simulink model "Balancing_Robot_Rob_Tracking"  (R2024b)
settings: Solver=VariableStepAuto  StartTime=0.0  StopTime=30  RelTol=1e-3
undefined symbols (not defined in the file): body, C12, C_filter, DiscIntNeverNeededParam, drv, dspblkCoreblockFVToolHelper, Fv_pr, g, g22, gbox, gcbh, K_Rob_LQR, Ki_calc, M11, M12_const, M22, mot, ms22g, Nu, Nx, sens, T, ua2tau, wheel
settings Model: Creator=liliy  LastModifiedBy=liliy

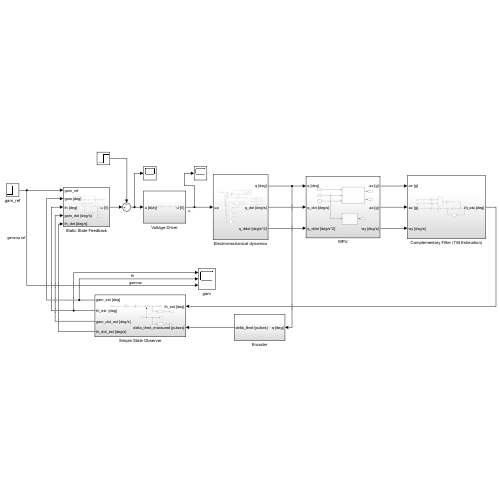
[thumbnail: Simulink's stored preview of the top-level diagram]
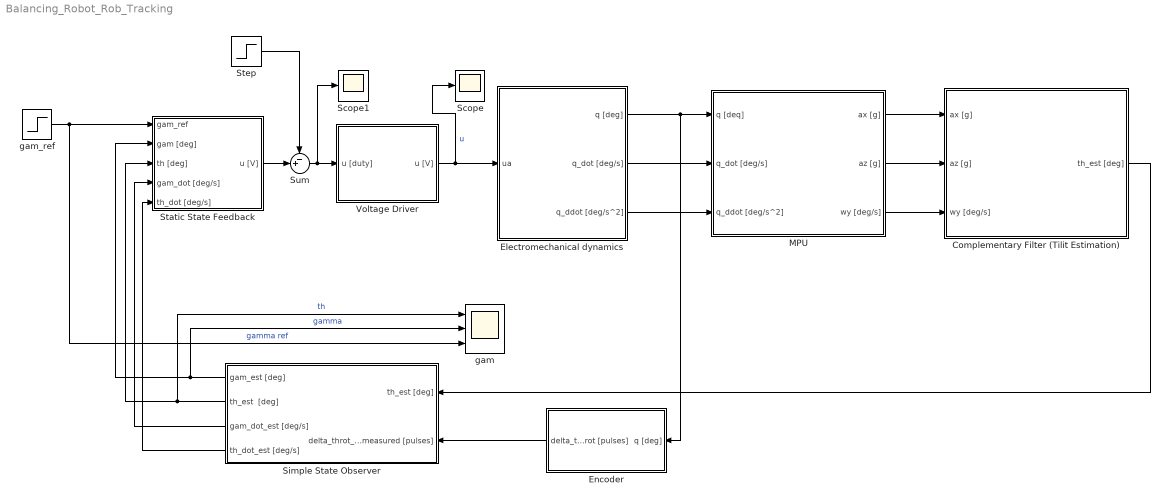
== system Balancing_Robot_Rob_Tracking ==
  Complementary Filter (Tilit Estimation) : Subsystem
  Electromechanical dynamics : Subsystem
  Encoder : Subsystem
  MPU : Subsystem
  Scope : Scope
  Scope1 : Scope
  Simple State Observer : Subsystem
  Static State Feedback : Subsystem
  Step : Step  Time=10  After=5/drv.duty2V  SampleTime=0
  Sum : Sum  Inputs=-+|
  Voltage Driver : Subsystem
  gam : Scope  NumInputPorts=3
  gam_ref : Step  Time=0  After=0.1/wheel.r*rad2deg  SampleTime=0
  wires:
  Voltage Driver/1(u [V]) -> Scope/1, Electromechanical dynamics/1(ua)  "u"
  Electromechanical dynamics/1(q [deg]) -> Encoder/1(q [deg]), MPU/1(q [deq])
  Electromechanical dynamics/2(q_dot [deg/s]) -> MPU/2(q_dot [deg/s])
  Electromechanical dynamics/3(q_ddot [deg/s^2]) -> MPU/3(q_ddot [deg/s^2])
  MPU/1(ax [g]) -> Complementary Filter (Tilit Estimation)/1(ax [g])
  MPU/2(az [g]) -> Complementary Filter (Tilit Estimation)/2(az [g])
  MPU/3(wy [deg/s]) -> Complementary Filter (Tilit Estimation)/3(wy [deg/s])
  Encoder/1(delta_throt [pulses]) -> Simple State Observer/2(delta_throt_measured [pulses])
  Complementary Filter (Tilit Estimation)/1(th_est [deg]) -> Simple State Observer/1(th_est [deg])
  Simple State Observer/1(gam_est [deg]) -> gam/2, Static State Feedback/2(gam [deg])  "gamma"
  Simple State Observer/2(th_est  [deg]) -> gam/1, Static State Feedback/3(th [deg])  "th"
  Simple State Observer/3(gam_dot_est [deg/s]) -> Static State Feedback/4(gam_dot [deg/s])
  Simple State Observer/4(th_dot_est [deg/s]) -> Static State Feedback/5(th_dot [deg/s])
  gam_ref/1 -> gam/3, Static State Feedback/1(gam_ref)  "gamma ref"
  Static State Feedback/1(u [V]) -> Sum/2
  Sum/1 -> Scope1/1, Voltage Driver/1(u [duty])
  Step/1 -> Sum/1

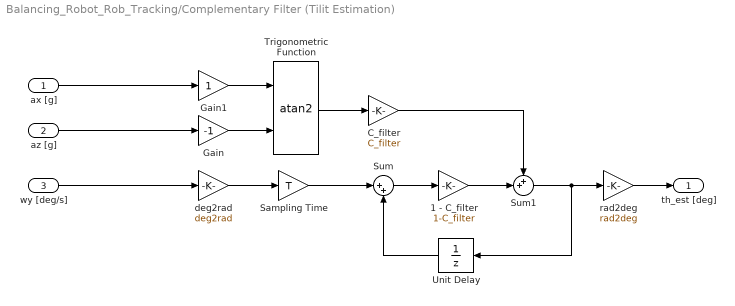
== system Balancing_Robot_Rob_Tracking/Complementary Filter (Tilit Estimation) ==
  ax [g] : Inport
  az [g] : Inport  Port=2
  wy [deg/s] : Inport  Port=3
  1 - C_filter : Gain  Gain=1-C_filter
  C_filter : Gain  Gain=C_filter
  Gain : Gain  Gain=-1
  Gain1 : Gain
  Sampling Time : Gain  Gain=T
  Sum : Sum  Inputs=|++
  Sum1 : Sum  Inputs=++|
  Trigonometric Function : Trigonometry  Operator=atan2
  Unit Delay : UnitDelay  SampleTime=T  HasFrameUpgradeWarning=on
  deg2rad : Gain  Gain=deg2rad
  rad2deg : Gain  Gain=rad2deg
  th_est [deg] : Outport
  wires:
  Trigonometric Function/1 -> C_filter/1
  Gain/1 -> Trigonometric Function/2
  rad2deg/1 -> th_est [deg]/1
  deg2rad/1 -> Sampling Time/1
  Sum/1 -> 1 - C_filter/1
  Gain1/1 -> Trigonometric Function/1
  Sum1/1 -> Unit Delay/1, rad2deg/1
  Sampling Time/1 -> Sum/1
  1 - C_filter/1 -> Sum1/2
  Unit Delay/1 -> Sum/2
  C_filter/1 -> Sum1/1
  ax [g]/1 -> Gain1/1
  az [g]/1 -> Gain/1
  wy [deg/s]/1 -> deg2rad/1

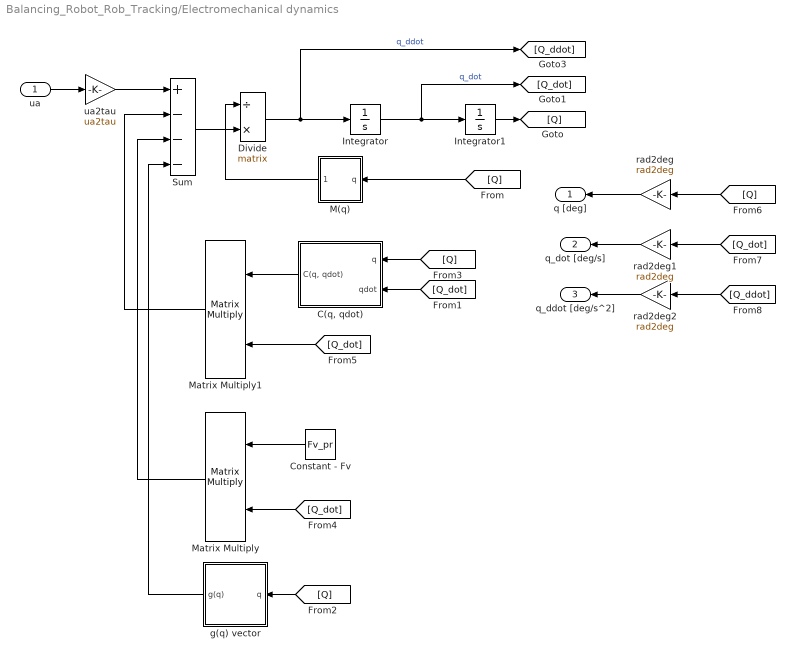
== system Balancing_Robot_Rob_Tracking/Electromechanical dynamics ==
  ua : Inport
  "C(q, qdot)" : Subsystem
  Constant - Fv : Constant  Value=Fv_pr
  Divide : Product  Inputs=/*  Multiplication=Matrix(*)
  Integrator : Integrator
  Integrator1 : Integrator
  M(q) : Subsystem
  Matrix Multiply : Product  Multiplication=Matrix(*)
  Matrix Multiply1 : Product  Multiplication=Matrix(*)
  Sum : Sum  Inputs=+---
  g(q) vector : Subsystem
  rad2deg : Gain  Gain=rad2deg
  rad2deg1 : Gain  Gain=rad2deg
  rad2deg2 : Gain  Gain=rad2deg
  ua2tau : Gain  Gain=ua2tau
  q [deg] : Outport
  q_dot [deg/s] : Outport  Port=2
  q_ddot [deg/s^2] : Outport  Port=3
  wires:
  [Q_dot] -> Matrix Multiply/2
  Integrator1/1 -> [Q]
  [Q] -> rad2deg/1
  [Q] -> M(q)/1(q)
  [Q_dot] -> "C(q, qdot)"/2(qdot)
  Divide/1 -> [Q_ddot], Integrator/1  "q_ddot"
  rad2deg1/1 -> q_dot [deg/s]/1
  Constant - Fv/1 -> Matrix Multiply/1
  ua2tau/1 -> Sum/1
  [Q_dot] -> Matrix Multiply1/2
  g(q) vector/1(g(q)) -> Sum/4
  Sum/1 -> Divide/2
  Matrix Multiply/1 -> Sum/3
  [Q] -> "C(q, qdot)"/1(q)
  [Q] -> g(q) vector/1(q)
  M(q)/1(M(q)) -> Divide/1
  "C(q, qdot)"/1("C(q, qdot)") -> Matrix Multiply1/1
  Integrator/1 -> Integrator1/1, [Q_dot]  "q_dot"
  Matrix Multiply1/1 -> Sum/2
  [Q_ddot] -> rad2deg2/1
  rad2deg/1 -> q [deg]/1
  [Q_dot] -> rad2deg1/1
  rad2deg2/1 -> q_ddot [deg/s^2]/1
  ua/1 -> ua2tau/1

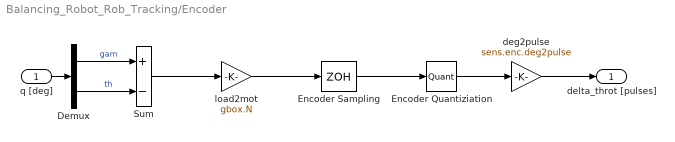
== system Balancing_Robot_Rob_Tracking/Encoder ==
  q [deg] : Inport
  Demux : Demux  Outputs=2
  Encoder Quantiziation : Quantizer  QuantizationInterval=sens.enc.pulse2deg
  Encoder Sampling : ZeroOrderHold  SampleTime=T
  Sum : Sum  Inputs=+-
  deg2pulse : Gain  Gain=sens.enc.deg2pulse
  load2mot : Gain  Gain=gbox.N
  delta_throt [pulses] : Outport
  wires:
  Demux/1 -> Sum/1  "gam"
  load2mot/1 -> Encoder Sampling/1
  Demux/2 -> Sum/2  "th"
  Encoder Sampling/1 -> Encoder Quantiziation/1
  deg2pulse/1 -> delta_throt [pulses]/1
  Encoder Quantiziation/1 -> deg2pulse/1
  Sum/1 -> load2mot/1
  q [deg]/1 -> Demux/1

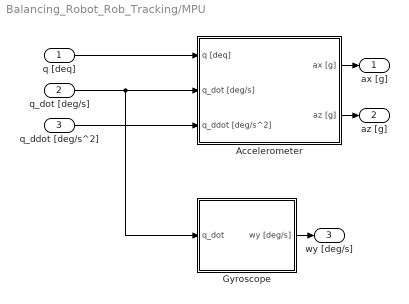
== system Balancing_Robot_Rob_Tracking/MPU ==
  q [deq] : Inport
  q_dot [deg/s] : Inport  Port=2
  q_ddot [deg/s^2] : Inport  Port=3
  Accelerometer : Subsystem
  Gyroscope : Subsystem
  ax [g] : Outport
  az [g] : Outport  Port=2
  wy [deg/s] : Outport  Port=3
  wires:
  Gyroscope/1(wy [deg/s]) -> wy [deg/s]/1
  q [deq]/1 -> Accelerometer/1(q [deq])
  Accelerometer/1(ax [g]) -> ax [g]/1
  Accelerometer/2(az [g]) -> az [g]/1
  q_dot [deg/s]/1 -> Gyroscope/1(q_dot), Accelerometer/2(q_dot [deg/s])
  q_ddot [deg/s^2]/1 -> Accelerometer/3(q_ddot [deg/s^2])

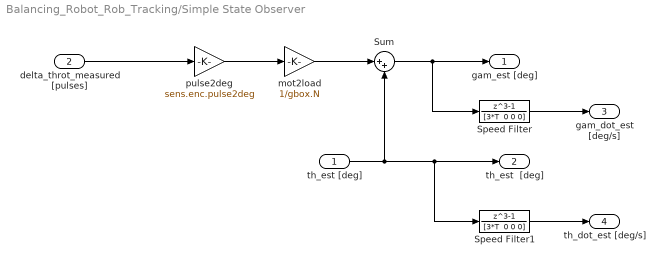
== system Balancing_Robot_Rob_Tracking/Simple State Observer ==
  th_est [deg] : Inport
  delta_throt_measured [pulses] : Inport  Port=2
  Speed Filter : DiscreteTransferFcn  LoadFcn=dspblkCoreblockFVToolHelper(gcbh,'load');  Numerator=[1 0 0 -1]  Denominator="[3*T  0 0 0]"
      settings: CopyFcn=dspblkCoreblockFVToolHelper(gcbh,'copy');  DeleteFcn=dspblkCoreblockFVToolHelper(gcbh,'close');  ModelCloseFcn=dspblkCoreblockFVToolHelper(gcbh,'close');  PreSaveFcn=dspblkCoreblockFVToolHelper(gcbh,'presave');  PostSaveFcn=dspblkCoreblockFVToolHelper(gcbh,'postsave');  CloseFcn=dspblkCoreblockFVToolHelper(gcbh,'close');
  Speed Filter1 : DiscreteTransferFcn  LoadFcn=dspblkCoreblockFVToolHelper(gcbh,'load');  Numerator=[1 0 0 -1]  Denominator="[3*T  0 0 0]"
      settings: CopyFcn=dspblkCoreblockFVToolHelper(gcbh,'copy');  DeleteFcn=dspblkCoreblockFVToolHelper(gcbh,'close');  ModelCloseFcn=dspblkCoreblockFVToolHelper(gcbh,'close');  PreSaveFcn=dspblkCoreblockFVToolHelper(gcbh,'presave');  PostSaveFcn=dspblkCoreblockFVToolHelper(gcbh,'postsave');  CloseFcn=dspblkCoreblockFVToolHelper(gcbh,'close');
  Sum : Sum  Inputs=|++
  mot2load : Gain  Gain=1/gbox.N
  pulse2deg : Gain  Gain=sens.enc.pulse2deg
  gam_est [deg] : Outport
  th_est  [deg] : Outport  Port=2
  gam_dot_est [deg/s] : Outport  Port=3
  th_dot_est [deg/s] : Outport  Port=4
  wires:
  Sum/1 -> Speed Filter/1, gam_est [deg]/1
  pulse2deg/1 -> mot2load/1
  Speed Filter/1 -> gam_dot_est [deg/s]/1
  delta_throt_measured [pulses]/1 -> pulse2deg/1
  Speed Filter1/1 -> th_dot_est [deg/s]/1
  th_est [deg]/1 -> Sum/2, Speed Filter1/1, th_est  [deg]/1
  mot2load/1 -> Sum/1

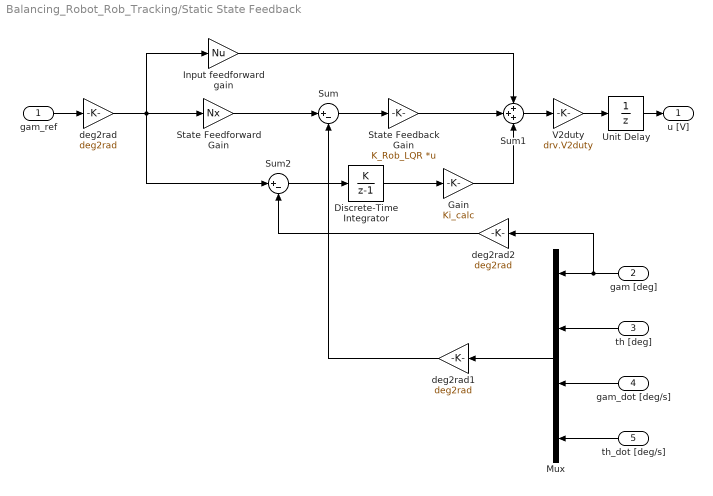
== system Balancing_Robot_Rob_Tracking/Static State Feedback ==
  gam_ref : Inport
  gam [deg] : Inport  Port=2
  th [deg] : Inport  Port=3
  gam_dot [deg/s] : Inport  Port=4
  th_dot [deg/s] : Inport  Port=5
  Discrete-Time Integrator : DiscreteIntegrator  IntegratorMethod=Accumulation: Forward Euler  SampleTime=T  ICPrevOutput=DiscIntNeverNeededParam  ICPrevScaledInput=DiscIntNeverNeededParam
  Gain : Gain  Gain=Ki_calc
  Input feedforward gain : Gain  Gain=Nu
  Mux : Mux
  State Feedback Gain : Gain  Gain=K_Rob_LQR  Multiplication=Matrix(K*u)
  State Feedforward Gain : Gain  Gain=Nx
  Sum : Sum  Inputs=|+-
  Sum1 : Sum  Inputs=+++
  Sum2 : Sum  Inputs=|+-
  Unit Delay : UnitDelay  SampleTime=T  HasFrameUpgradeWarning=on
  V2duty : Gain  Gain=drv.V2duty
  deg2rad : Gain  Gain=deg2rad
  deg2rad1 : Gain  Gain=deg2rad
  deg2rad2 : Gain  Gain=deg2rad
  u [V] : Outport
  wires:
  gam_ref/1 -> deg2rad/1
  deg2rad/1 -> Sum2/1, State Feedforward Gain/1, Input feedforward gain/1
  State Feedforward Gain/1 -> Sum/1
  Sum/1 -> State Feedback Gain/1
  State Feedback Gain/1 -> Sum1/2
  Input feedforward gain/1 -> Sum1/1
  Sum1/1 -> V2duty/1
  Mux/1 -> deg2rad1/1
  gam_dot [deg/s]/1 -> Mux/3
  th_dot [deg/s]/1 -> Mux/4
  V2duty/1 -> Unit Delay/1
  gam [deg]/1 -> deg2rad2/1, Mux/1
  th [deg]/1 -> Mux/2
  deg2rad1/1 -> Sum/2
  Unit Delay/1 -> u [V]/1
  deg2rad2/1 -> Sum2/2
  Sum2/1 -> Discrete-Time Integrator/1
  Discrete-Time Integrator/1 -> Gain/1
  Gain/1 -> Sum1/3

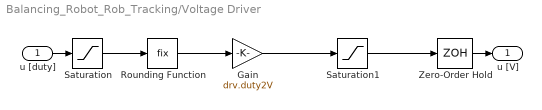
== system Balancing_Robot_Rob_Tracking/Voltage Driver ==
  u [duty] : Inport
  Gain : Gain  Gain=drv.duty2V
  Rounding Function : Rounding  Operator=fix
  Saturation : Saturate  UpperLimit=drv.dutymax  LowerLimit=-drv.dutymax
  Saturation1 : Saturate  UpperLimit=drv.Vbus  LowerLimit=-drv.Vbus
  Zero-Order Hold : ZeroOrderHold  SampleTime=T
  u [V] : Outport
  wires:
  Saturation/1 -> Rounding Function/1
  u [duty]/1 -> Saturation/1
  Zero-Order Hold/1 -> u [V]/1
  Saturation1/1 -> Zero-Order Hold/1
  Rounding Function/1 -> Gain/1
  Gain/1 -> Saturation1/1

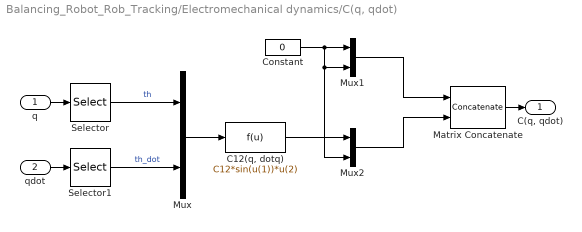
== system Balancing_Robot_Rob_Tracking/Electromechanical dynamics/C(q, qdot) ==
  q : Inport
  qdot : Inport  Port=2
  "C12(q, dotq)" : Fcn  Expr=C12*sin(u(1))*u(2)
  Constant : Constant  Value=0
  Matrix Concatenate : Concatenate  Mode=Multidimensional array  ConcatenateDimension=2
  Mux : Mux  Inputs=2
  Mux1 : Mux  Inputs=2
  Mux2 : Mux  Inputs=2
  Selector : Selector  InputPortWidth=2  IndexOptions=Index vector (dialog)  Indices=[2]  OutputSizes=1
  Selector1 : Selector  InputPortWidth=2  IndexOptions=Index vector (dialog)  Indices=[2]  OutputSizes=1
  "C(q, qdot)" : Outport
  wires:
  Mux/1 -> "C12(q, dotq)"/1
  Selector1/1 -> Mux/2  "th_dot"
  Mux2/1 -> Matrix Concatenate/2
  Constant/1 -> Mux2/2, Mux1/2, Mux1/1
  Selector/1 -> Mux/1  "th"
  "C12(q, dotq)"/1 -> Mux2/1
  Mux1/1 -> Matrix Concatenate/1
  qdot/1 -> Selector1/1
  Matrix Concatenate/1 -> "C(q, qdot)"/1
  q/1 -> Selector/1

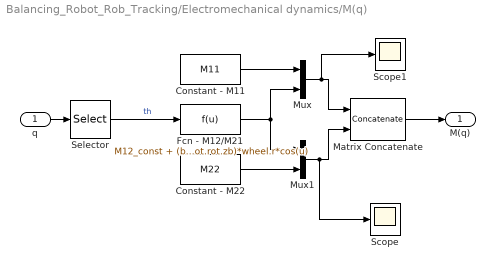
== system Balancing_Robot_Rob_Tracking/Electromechanical dynamics/M(q) ==
  q : Inport
  Constant - M11 : Constant  Value=M11
  Constant - M22 : Constant  Value=M22
  Fcn - M12/M21 : Fcn  Expr=M12_const + (body.m*body.zb + 2*mot.rot.m*mot.rot.zb)*wheel.r*cos(u)
  Matrix Concatenate : Concatenate  Mode=Multidimensional array  ConcatenateDimension=2
  Mux : Mux  Inputs=2
  Mux1 : Mux  Inputs=2
  Scope : Scope
  Scope1 : Scope
  Selector : Selector  InputPortWidth=2  IndexOptions=Index vector (dialog)  Indices=[2]  OutputSizes=1
  M(q) : Outport
  wires:
  q/1 -> Selector/1
  Selector/1 -> Fcn - M12/M21/1  "th"
  Fcn - M12/M21/1 -> Mux/2, Mux1/1
  Constant - M22/1 -> Mux1/2
  Constant - M11/1 -> Mux/1
  Mux/1 -> Scope1/1, Matrix Concatenate/1
  Mux1/1 -> Scope/1, Matrix Concatenate/2
  Matrix Concatenate/1 -> M(q)/1

== system Balancing_Robot_Rob_Tracking/Electromechanical dynamics/g(q) vector ==
  q : Inport
  Constant : Constant  Value=0
  Fcn-g2(q) : Fcn  Expr=g22*sin(u)
  Mux : Mux  Inputs=2
  Selector : Selector  InputPortWidth=2  IndexOptions=Index vector (dialog)  Indices=[2]  OutputSizes=1
  g(q) : Outport
  wires:
  q/1 -> Selector/1
  Selector/1 -> Fcn-g2(q)/1  "th"
  Fcn-g2(q)/1 -> Mux/2
  Mux/1 -> g(q)/1
  Constant/1 -> Mux/1

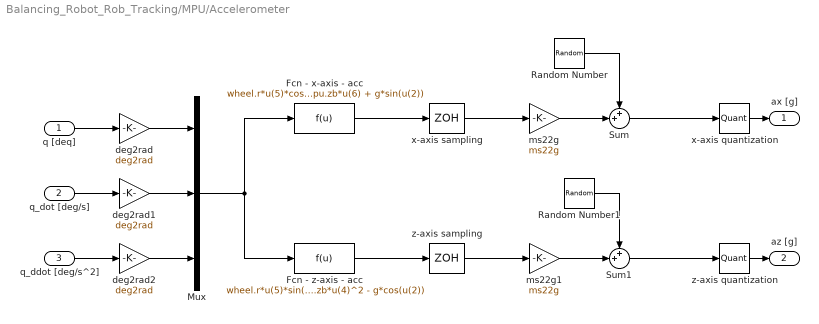
== system Balancing_Robot_Rob_Tracking/MPU/Accelerometer ==
  q [deq] : Inport
  q_dot [deg/s] : Inport  Port=2
  q_ddot [deg/s^2] : Inport  Port=3
  Fcn - x-axis - acc : Fcn  Expr=wheel.r*u(5)*cos(u(2)) + sens.mpu.zb*u(6) + g*sin(u(2))
  Fcn - z-axis - acc : Fcn  Expr=wheel.r*u(5)*sin(u(2)) - sens.mpu.zb*u(4)^2 - g*cos(u(2))
  Mux : Mux  Inputs=3
  Random Number : RandomNumber  Variance=sens.mpu.acc.noisevar  SampleTime=T
  Random Number1 : RandomNumber  Variance=sens.mpu.acc.noisevar  SampleTime=T
  Sum : Sum  Inputs=++|
  Sum1 : Sum  Inputs=++|
  deg2rad : Gain  Gain=deg2rad
  deg2rad1 : Gain  Gain=deg2rad
  deg2rad2 : Gain  Gain=deg2rad
  ms22g : Gain  Gain=ms22g
  ms22g1 : Gain  Gain=ms22g
  x-axis quantization : Quantizer  QuantizationInterval=sens.mpu.acc.LSB2g
  x-axis sampling : ZeroOrderHold  SampleTime=T
  z-axis quantization : Quantizer  QuantizationInterval=sens.mpu.acc.LSB2g
  z-axis sampling : ZeroOrderHold  SampleTime=T
  ax [g] : Outport
  az [g] : Outport  Port=2
  wires:
  Random Number/1 -> Sum/1
  Sum/1 -> x-axis quantization/1
  Mux/1 -> Fcn - z-axis - acc/1, Fcn - x-axis - acc/1
  Sum1/1 -> z-axis quantization/1
  deg2rad1/1 -> Mux/2
  Random Number1/1 -> Sum1/1
  ms22g/1 -> Sum/2
  deg2rad2/1 -> Mux/3
  Fcn - z-axis - acc/1 -> z-axis sampling/1
  Fcn - x-axis - acc/1 -> x-axis sampling/1
  deg2rad/1 -> Mux/1
  z-axis sampling/1 -> ms22g1/1
  ms22g1/1 -> Sum1/2
  x-axis sampling/1 -> ms22g/1
  x-axis quantization/1 -> ax [g]/1
  z-axis quantization/1 -> az [g]/1
  q [deq]/1 -> deg2rad/1
  q_ddot [deg/s^2]/1 -> deg2rad2/1
  q_dot [deg/s]/1 -> deg2rad1/1

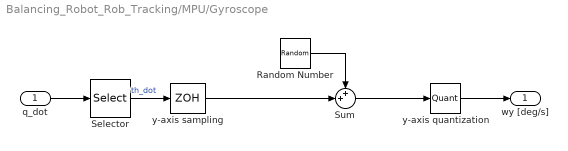
== system Balancing_Robot_Rob_Tracking/MPU/Gyroscope ==
  q_dot : Inport
  Random Number : RandomNumber  Variance=sens.mpu.gyro.noisevar  SampleTime=T
  Selector : Selector  InputPortWidth=2  IndexOptions=Index vector (dialog)  Indices=[2]  OutputSizes=1
  Sum : Sum  Inputs=++|
  y-axis quantization : Quantizer  QuantizationInterval=sens.mpu.gyro.LSB2degs
  y-axis sampling : ZeroOrderHold  SampleTime=T
  wy [deg/s] : Outport
  wires:
  y-axis quantization/1 -> wy [deg/s]/1
  Random Number/1 -> Sum/1
  q_dot/1 -> Selector/1
  y-axis sampling/1 -> Sum/2
  Sum/1 -> y-axis quantization/1
  Selector/1 -> y-axis sampling/1  "th_dot"
